simulink subsystem "BatteryHV_BasicThermal_refsub"  (R2026a)
settings: Solver=VariableStepAuto
PreLoadFcn:
  | defineBus_HighVoltage
undefined symbols (not defined in the file or in its folder): batteryHV, initial, Minus, Plus
libraries: fl_lib x20, nesl_utility x9, sdl_lib x1
settings Model: Creator=isaacito  LastModifiedBy=isaacito
settings SimscapeCC: SimscapeNominalValues="[{\"value\":\"1\",\"unit\":\"A\"},{\"value\":\"1\",\"unit\":\"bar\"},{\"value\":\"1\",\"unit\":\"cm^2\"},{\"value\":\"1\",\"unit\":\"cm^3/s\"},{\"value\":\"1\",\"unit\":\"kJ/kg\"},{\"value\":\"1\",\"unit\":\"kW\"},{\"value\":\"1\",\"unit\":\"l\"},{\"value\":\"1\",\"unit\":\"N\"},{\"value\":\"1\",\"unit\":\"N*m\"},{\"value\":\"1\",\"unit\":\"V\"}]"  SimscapeLogType=none  SimscapeLogDataHistory=5000.0

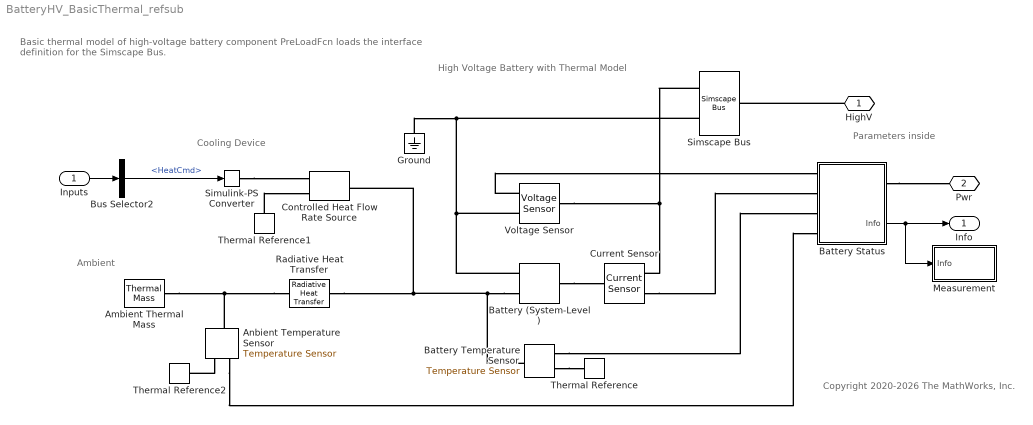
== system BatteryHV_BasicThermal_refsub ==
  note: High Voltage Battery with Thermal Model
  note: Cooling Device
  note: Ambient
  note: Copyright 2020-2026 The MathWorks, Inc.
  note: Parameters inside
  note: Basic thermal model of high-voltage battery component
      | PreLoadFcn loads the interface definition for the Simscape Bus.
  Inputs : Inport
  Ambient Thermal Mass : fl_lib/Thermal/Thermal Elements/Thermal Mass  mass_type=foundation.enum.constant_variable.constant  mass=batteryHV.ambientMass_t t  sp_heat=batteryHV.ambientSpecificHeat_J_per_Kkg J/(K*kg)  mass_min=1e-6 kg  num_ports=foundation.enum.numPorts2.one  m_specify=off  m_priority=High  m=1 kg  m_nominal_specify=off  m_nominal_value=1  m_nominal_unit=kg  T_specify=on  T_priority=High  T=initial.ambientTemp_K K  T_nominal_specify=off  T_nominal_value=1  T_nominal_unit=K  Q_specify=off  Q_priority=None  Q=0 W  Q_nominal_specify=off  Q_nominal_value=1  Q_nominal_unit=W
  Anbient Temperature Sensor : fl_lib/Thermal/Thermal Sensors/Temperature Sensor  temperature_measure=foundation.enum.MeasurementReference.difference
  Battery (System-Level) : sdl_lib/Sources/Battery (System-Level)  Vnom=batteryHV.nominalVoltage_V V  R1=batteryHV.internalResistance_Ohm Ohm  prm_AH=sdl.enum.InfiniteFinite.Finite  AH=batteryHV.nominalCharge_Ahr A*hr  V1=batteryHV.measuredVoltage_V V  AH1=batteryHV.measuredCharge_Ahr A*hr  prm_R2=sdl.enum.DisabledEnabled.Disabled  R2=2000 Ohm  thermal_port=simscape.enum.thermaleffects.model  thermal_mass=batteryHV.ThermalMass_J_per_K J/K  i_specify=off  i_priority=None  i=0 A  i_nominal_specify=off  i_nominal_value=1  i_nominal_unit=A  v_specify=off  v_priority=None  v=0 V  v_nominal_specify=off  v_nominal_value=1  v_nominal_unit=V  charge_specify=on  charge_priority=High  charge=initial.hvBattery_Charge_Ahr A*hr  charge_nominal_specify=off  charge_nominal_value=1  charge_nominal_unit=A*hr  temperature_specify=on  temperature_priority=High  temperature=initial.hvBattery_Temperature_K K  temperature_nominal_specify=off  temperature_nominal_value=1  temperature_nominal_unit=K
  Battery Status : Subsystem
      settings: PortSchema="{\"entries\":[{\"content\":{\"sides\":[{\"content\":{\"connectorIds\":[\"LConn1\",\"LConn2\",\"LConn3\",\"LConn4\"]},\"type\":\"ConnectorPlacement.EquallySpacedRectSide\",\"uuid\":\"2ad7e292-de4e-4a00-bc26-5f2422ad78d1\"},{\"content\":{\"connectorIds\":[\"RConn1\",\"Out1\"],\"side\":\"RIGHT\"},\"type\":\"ConnectorPlacement.EquallySpacedRectSide\",\"uuid\":\"34d8611e-8b74-4415-b778-0d39f0867232\"},{\"content\":{\"side\":\"TOP\"},\"type\":\"ConnectorPlacement.EquallySpacedRectSide\",\"uuid\":\"1cae1697-d501-4f4c-9a8a-53bb589c31c8\"}]},\"type\":\"ConnectorPlacement.EquallySpacedConnector\",\"uuid\":\"7ded3142-d61d-4aa2-80a2-3b88c0fe4f70\"}],\"packageUris\":[\"http://schema.mathworks.com/mf0/Connector/R2020b\"],\"version\":\"1.0\"}"
  Battery Temperature Sensor : fl_lib/Thermal/Thermal Sensors/Temperature Sensor  temperature_measure=foundation.enum.MeasurementReference.difference
  Bus Selector2 : BusSelector  OutputSignals=HeatCmd
  Controlled Heat Flow Rate Source : fl_lib/Thermal/Thermal Sources/Controlled Heat Flow Rate Source
  Current Sensor : fl_lib/Electrical/Electrical Sensors/Current Sensor
  Ground : fl_lib/Electrical/Electrical Elements/Electrical Reference
  Measurement : Subsystem
  Radiative Heat Transfer : fl_lib/Thermal/Thermal Elements/Radiative Heat Transfer  area=batteryHV.RadiationArea_m2 m^2  rad_tr_coeff=batteryHV.RadiationCoeff_W_per_K4m2 W/(K^4*m^2)  T_specify=off  T_priority=None  T=0 K  T_nominal_specify=off  T_nominal_value=1  T_nominal_unit=K  Q_specify=off  Q_priority=None  Q=0 W  Q_nominal_specify=off  Q_nominal_value=1  Q_nominal_unit=W
  Simscape Bus : SimscapeBus  HierarchyStrings=Plus;Minus  ConnectionType=Bus: Bus_HighVoltage
      settings: AttributesFormatString=%<ConnectionType>
  Simulink-PS Converter : nesl_utility/Simulink-PS Converter  PhysicalDomain=network_engine_domain  SubClassName=ps_input  LeftPortType=input  RightPortType=output  PseudoPeriodic=off  Frequencies=[]  NoiseDistribution=none  NoiseParameters=[]  Unit=W  AffineConversion=off  FilteringAndDerivatives=provide  SimscapeFilterOrder=1  InputFilterTimeConstant=0.001  UdotUserProvided=0
  Thermal Reference : fl_lib/Thermal/Thermal Elements/Thermal Reference
  Thermal Reference1 : fl_lib/Thermal/Thermal Elements/Thermal Reference
  Thermal Reference2 : fl_lib/Thermal/Thermal Elements/Thermal Reference
  Voltage Sensor : fl_lib/Electrical/Electrical Sensors/Voltage Sensor
  HighV : PMIOPort  Side=Right
  Pwr : PMIOPort  Port=2  Side=Right
  Info : Outport
  wires:
  Battery Status/1(Info) -> Info/1, Measurement/1(Info)
  Inputs/1 -> Bus Selector2/1
  Bus Selector2/1 -> Simulink-PS Converter/1  "<HeatCmd>"
  connections:
  Battery (System-Level)/RConn1 -- Voltage Sensor/RConn2 -- Ground/LConn1 -- Simscape Bus/LConn2
  Voltage Sensor/LConn1 -- Simscape Bus/LConn1 -- Current Sensor/RConn2
  Battery (System-Level)/RConn2 -- Controlled Heat Flow Rate Source/LConn1 -- Radiative Heat Transfer/RConn1 -- Battery Temperature Sensor/LConn1
  Radiative Heat Transfer/LConn1 -- Anbient Temperature Sensor/LConn1 -- Ambient Thermal Mass/LConn1
  Current Sensor/RConn1 -- Battery Status/LConn2
  Voltage Sensor/RConn1 -- Battery Status/LConn1
  HighV/RConn1 -- Simscape Bus/RConn1
  Battery (System-Level)/LConn1 -- Current Sensor/LConn1
  Battery Temperature Sensor/RConn2 -- Battery Status/LConn3
  Thermal Reference1/LConn1 -- Controlled Heat Flow Rate Source/RConn2
  Simulink-PS Converter/RConn1 -- Controlled Heat Flow Rate Source/RConn1
  Battery Temperature Sensor/RConn1 -- Thermal Reference/LConn1
  Anbient Temperature Sensor/RConn1 -- Thermal Reference2/LConn1
  Anbient Temperature Sensor/RConn2 -- Battery Status/LConn4
  Battery Status/RConn1 -- Pwr/RConn1

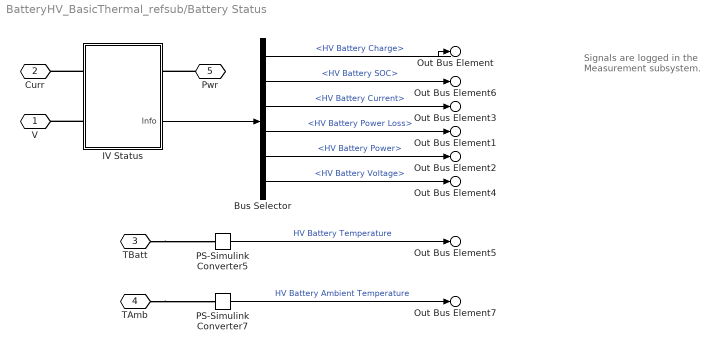
== system BatteryHV_BasicThermal_refsub/Battery Status ==
  note: Signals are logged in
      | the Measurement subsystem.
  Bus Selector : BusSelector  OutputSignals=HV Battery Charge,HV Battery SOC,HV Battery Current,HV Battery Power Loss,HV Battery Power,HV Battery Voltage
  IV Status : Subsystem
      settings: PortSchema="{\"entries\":[{\"content\":{\"sides\":[{\"content\":{\"connectorIds\":[\"LConn1\",\"LConn2\"]},\"type\":\"ConnectorPlacement.EquallySpacedRectSide\",\"uuid\":\"fa3fe2c3-d9c0-40ca-976a-fdfa614694fc\"},{\"content\":{\"connectorIds\":[\"RConn1\",\"Out1\"],\"side\":\"RIGHT\"},\"type\":\"ConnectorPlacement.EquallySpacedRectSide\",\"uuid\":\"d6ed96ef-770b-4a18-8b31-ef7e8f253069\"},{\"content\":{\"side\":\"TOP\"},\"type\":\"ConnectorPlacement.EquallySpacedRectSide\",\"uuid\":\"d9a8161e-0196-4518-8226-4ae50c8bd457\"}]},\"type\":\"ConnectorPlacement.EquallySpacedConnector\",\"uuid\":\"0aac0953-a631-4fd0-93f3-a84e629f2b58\"}],\"packageUris\":[\"http://schema.mathworks.com/mf0/Connector/R2020b\"],\"version\":\"1.0\"}"
  PS-Simulink Converter5 : nesl_utility/PS-Simulink Converter  PhysicalDomain=network_engine_domain  SubClassName=ps_output  LeftPortType=input  RightPortType=output  PseudoPeriodic=off  Frequencies=[]  VectorFormat=inherit  Unit=degC  AffineConversion=on
  PS-Simulink Converter7 : nesl_utility/PS-Simulink Converter  PhysicalDomain=network_engine_domain  SubClassName=ps_output  LeftPortType=input  RightPortType=output  PseudoPeriodic=off  Frequencies=[]  VectorFormat=inherit  Unit=degC  AffineConversion=on
  V : PMIOPort  Side=Left
  Curr : PMIOPort  Port=2  Side=Left
  TBatt : PMIOPort  Port=3  Side=Left
  TAmb : PMIOPort  Port=4  Side=Left
  Pwr : PMIOPort  Port=5  Side=Right
  Out Bus Element : Outport  PortName=Info  Element=Charge
  Out Bus Element3 : Outport  PortName=Info  Element=Current
  Out Bus Element1 : Outport  PortName=Info  Element=PowerLoss
  Out Bus Element2 : Outport  PortName=Info  Element=Power
  Out Bus Element4 : Outport  PortName=Info  Element=Voltage
  Out Bus Element5 : Outport  PortName=Info  Element=Temp
  Out Bus Element6 : Outport  PortName=Info  Element=SOC
  Out Bus Element7 : Outport  PortName=Info  Element=TempAmb
  wires:
  PS-Simulink Converter7/1 -> Out Bus Element7/1  "HV Battery Ambient Temperature"
  PS-Simulink Converter5/1 -> Out Bus Element5/1  "HV Battery Temperature"
  IV Status/1(Info) -> Bus Selector/1
  Bus Selector/1 -> Out Bus Element/1  "<HV Battery Charge>"
  Bus Selector/2 -> Out Bus Element6/1  "<HV Battery SOC>"
  Bus Selector/3 -> Out Bus Element3/1  "<HV Battery Current>"
  Bus Selector/4 -> Out Bus Element1/1  "<HV Battery Power Loss>"
  Bus Selector/5 -> Out Bus Element2/1  "<HV Battery Power>"
  Bus Selector/6 -> Out Bus Element4/1  "<HV Battery Voltage>"
  connections:
  TAmb/RConn1 -- PS-Simulink Converter7/LConn1
  TBatt/RConn1 -- PS-Simulink Converter5/LConn1
  IV Status/LConn1 -- Curr/RConn1
  IV Status/LConn2 -- V/RConn1
  Pwr/RConn1 -- IV Status/RConn1

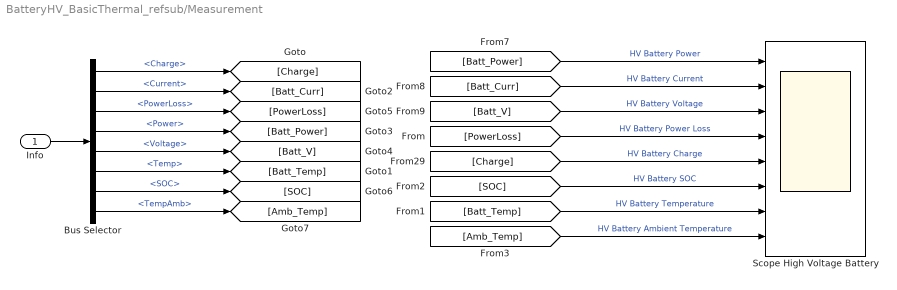
== system BatteryHV_BasicThermal_refsub/Measurement ==
  Info : Inport
  Bus Selector : BusSelector  OutputSignals=Charge,Current,PowerLoss,Power,Voltage,Temp,SOC,TempAmb
  Scope High Voltage Battery : Scope  NumInputPorts=8
      settings: ActiveDisplayYMinimum=-2.22148  ActiveDisplayYMaximum=4.24683
  wires:
  [SOC] -> Scope High Voltage Battery/6  "HV Battery SOC"
  [Amb_Temp] -> Scope High Voltage Battery/8  "HV Battery Ambient Temperature"
  [Batt_Temp] -> Scope High Voltage Battery/7  "HV Battery Temperature"
  Bus Selector/7 -> [SOC]  "<SOC>"
  [Charge] -> Scope High Voltage Battery/5  "HV Battery Charge"
  [PowerLoss] -> Scope High Voltage Battery/4  "HV Battery Power Loss"
  Bus Selector/2 -> [Batt_Curr]  "<Current>"
  Bus Selector/4 -> [Batt_Power]  "<Power>"
  [Batt_V] -> Scope High Voltage Battery/3  "HV Battery Voltage"
  Bus Selector/6 -> [Batt_Temp]  "<Temp>"
  [Batt_Power] -> Scope High Voltage Battery/1  "HV Battery Power"
  Bus Selector/8 -> [Amb_Temp]  "<TempAmb>"
  [Batt_Curr] -> Scope High Voltage Battery/2  "HV Battery Current"
  Bus Selector/5 -> [Batt_V]  "<Voltage>"
  Info/1 -> Bus Selector/1
  Bus Selector/3 -> [PowerLoss]  "<PowerLoss>"
  Bus Selector/1 -> [Charge]  "<Charge>"

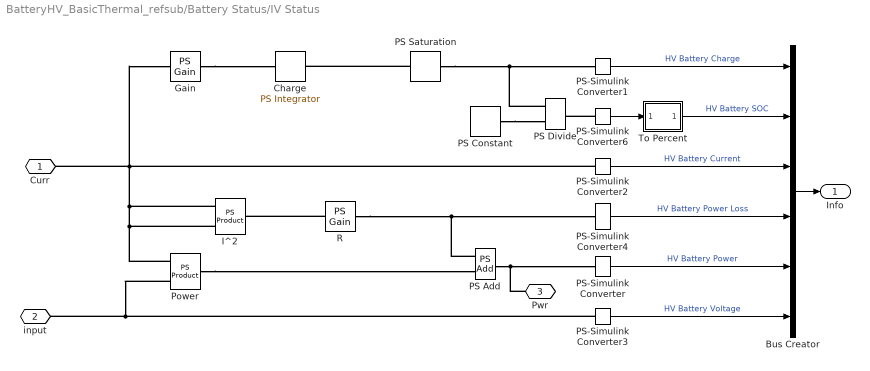
== system BatteryHV_BasicThermal_refsub/Battery Status/IV Status ==
  Bus Creator : BusCreator  Inputs=6
  Charge : fl_lib/Physical Signals/Linear Operators/PS Integrator  reset_method=foundation.enum.IntegratorResetSpec.None  initial_condition_spec=foundation.enum.IntegratorICSpec.Internal  saturation_spec=foundation.enum.IntegratorSaturationSpec.None  saturation_source_spec=foundation.enum.IntegratorSaturationSourceSpec.Internal  x0=initial.hvBattery_Charge_Ahr A*hr  xu=inf s  xl=-inf s
      settings: AttributesFormatString=%<x0> [%<x0_unit>]
  Gain : fl_lib/Physical Signals/Functions/PS Gain  gain=-1
      settings: AttributesFormatString=%<gain>
  I^2 : fl_lib/Physical Signals/Functions/PS Product
  PS Add : fl_lib/Physical Signals/Functions/PS Add
  PS Constant : fl_lib/Physical Signals/Sources/PS Constant  constant=batteryHV.nominalCharge_Ahr A*hr
      settings: AttributesFormatString=%<constant> [%<constant_unit>]
  PS Divide : fl_lib/Physical Signals/Functions/PS Divide
  PS Saturation : fl_lib/Physical Signals/Nonlinear Operators/PS Saturation  upper_limit=batteryHV.nominalCharge_Ahr A*hr  lower_limit=0 A*hr  ZeroCross=true
      settings: AttributesFormatString=|
      | Upper: %<upper_limit>
      | Lower: %<lower_limit>
  PS-Simulink Converter : nesl_utility/PS-Simulink Converter  PhysicalDomain=network_engine_domain  SubClassName=ps_output  LeftPortType=input  RightPortType=output  PseudoPeriodic=off  Frequencies=[]  VectorFormat=1-D array  Unit=kW  AffineConversion=off
  PS-Simulink Converter1 : nesl_utility/PS-Simulink Converter  PhysicalDomain=network_engine_domain  SubClassName=ps_output  LeftPortType=input  RightPortType=output  PseudoPeriodic=off  Frequencies=[]  VectorFormat=1-D array  Unit=A*hr  AffineConversion=off
  PS-Simulink Converter2 : nesl_utility/PS-Simulink Converter  PhysicalDomain=network_engine_domain  SubClassName=ps_output  LeftPortType=input  RightPortType=output  PseudoPeriodic=off  Frequencies=[]  VectorFormat=1-D array  Unit=A  AffineConversion=off
  PS-Simulink Converter3 : nesl_utility/PS-Simulink Converter  PhysicalDomain=network_engine_domain  SubClassName=ps_output  LeftPortType=input  RightPortType=output  PseudoPeriodic=off  Frequencies=[]  VectorFormat=1-D array  Unit=V  AffineConversion=off
  PS-Simulink Converter4 : nesl_utility/PS-Simulink Converter  PhysicalDomain=network_engine_domain  SubClassName=ps_output  LeftPortType=input  RightPortType=output  PseudoPeriodic=off  Frequencies=[]  VectorFormat=1-D array  Unit=W  AffineConversion=off
  PS-Simulink Converter6 : nesl_utility/PS-Simulink Converter  PhysicalDomain=network_engine_domain  SubClassName=ps_output  LeftPortType=input  RightPortType=output  PseudoPeriodic=off  Frequencies=[]  VectorFormat=1-D array  Unit=1  AffineConversion=off
  Power : fl_lib/Physical Signals/Functions/PS Product
  R : fl_lib/Physical Signals/Functions/PS Gain  gain=batteryHV.internalResistance_Ohm Ohm
      settings: AttributesFormatString=%<gain> [%<gain_unit>]
  To Percent : Subsystem
  Curr : PMIOPort  Side=Left
  input : PMIOPort  Port=2  Side=Left
  Pwr : PMIOPort  Port=3  Side=Right
  Info : Outport
  wires:
  To Percent/1(Out1) -> Bus Creator/2  "HV Battery SOC"
  PS-Simulink Converter4/1 -> Bus Creator/4  "HV Battery Power Loss"
  PS-Simulink Converter3/1 -> Bus Creator/6  "HV Battery Voltage"
  PS-Simulink Converter1/1 -> Bus Creator/1  "HV Battery Charge"
  PS-Simulink Converter6/1 -> To Percent/1(In1)
  PS-Simulink Converter2/1 -> Bus Creator/3  "HV Battery Current"
  PS-Simulink Converter/1 -> Bus Creator/5  "HV Battery Power"
  Bus Creator/1 -> Info/1
  connections:
  PS Add/RConn1 -- Pwr/RConn1 -- PS-Simulink Converter/LConn1
  Power/RConn1 -- PS Add/LConn2
  PS Saturation/LConn1 -- Charge/RConn1
  PS Divide/LConn1 -- PS-Simulink Converter1/LConn1 -- PS Saturation/RConn1
  Power/LConn2 -- I^2/LConn1 -- I^2/LConn2 -- PS-Simulink Converter2/LConn1 -- Gain/LConn1 -- Curr/RConn1
  Power/LConn1 -- PS-Simulink Converter3/LConn1 -- input/RConn1
  PS Constant/RConn1 -- PS Divide/LConn2
  Gain/RConn1 -- Charge/LConn1
  PS-Simulink Converter6/LConn1 -- PS Divide/RConn1
  R/LConn1 -- I^2/RConn1
  R/RConn1 -- PS-Simulink Converter4/LConn1 -- PS Add/LConn1

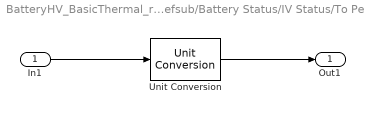
== system BatteryHV_BasicThermal_refsub/Battery Status/IV Status/To Percent ==
  In1 : Inport
  Unit Conversion : UnitConversion
  Out1 : Outport  Unit=%
      settings: AttributesFormatString=%<Unit>
  wires:
  In1/1 -> Unit Conversion/1
  Unit Conversion/1 -> Out1/1
